simulink model "RingSpinning_Bearing_DigitalTwin_Modely"  (R2025b)
settings: Solver=ode4  StartTime=0.0  StopTime=10  FixedStep=7.8125e-05  RelTol=1e-3
undefined symbols (not defined in the file): ambient_temp, bpfo_hz, Cth, damping_ratio, fault_severity, imbalance_amp, initial_temp, Kth, misalignment_amp, omega, P_loss, rpm, sensor_noise_std, wn
settings Model: Creator=Dhiyayanth  LastModifiedBy=Dhiyayanth

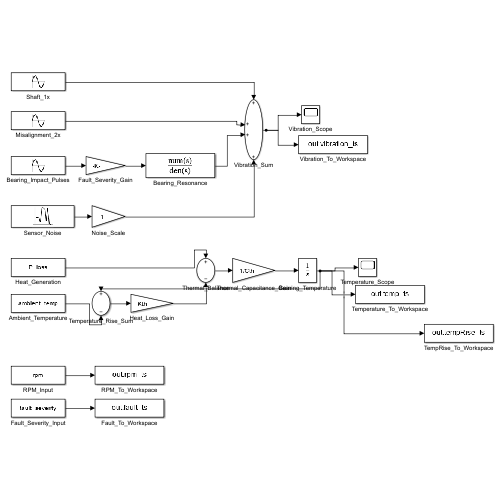
[thumbnail: Simulink's stored preview of the top-level diagram]
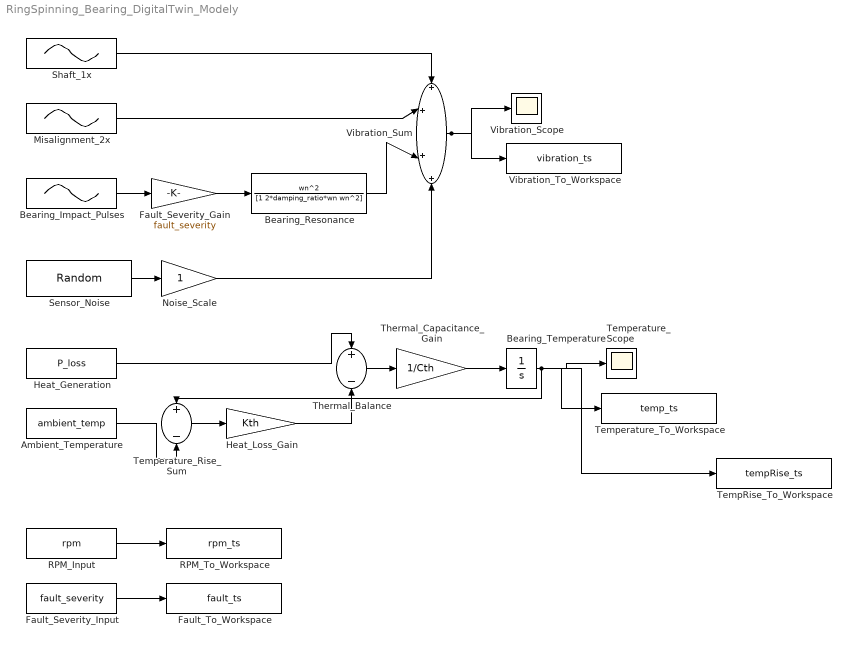
== system RingSpinning_Bearing_DigitalTwin_Modely ==
  Ambient_Temperature : Constant  Value=ambient_temp
  Bearing_Impact_Pulses : Sin  Frequency=2*pi*bpfo_hz  SampleTime=0
  Bearing_Resonance : TransferFcn  Numerator=wn^2  Denominator=[1 2*damping_ratio*wn wn^2]
  Bearing_Temperature : Integrator  InitialCondition=initial_temp
  Fault_Severity_Gain : Gain  Gain=fault_severity
  Fault_Severity_Input : Constant  Value=fault_severity
  Fault_To_Workspace : ToWorkspace  VariableName=fault_ts  SaveFormat=Timeseries  SampleTime=-1
  Heat_Generation : Constant  Value=P_loss
  Heat_Loss_Gain : Gain  Gain=Kth
  Misalignment_2x : Sin  Amplitude=misalignment_amp  Frequency=2*omega  SampleTime=0
  Noise_Scale : Gain
  RPM_Input : Constant  Value=rpm
  RPM_To_Workspace : ToWorkspace  VariableName=rpm_ts  SaveFormat=Timeseries  SampleTime=-1
  Sensor_Noise : RandomNumber  Variance=sensor_noise_std^2  Seed=1234  SampleTime=7.8125e-05
  Shaft_1x : Sin  Amplitude=imbalance_amp  Frequency=omega  SampleTime=0
  TempRise_To_Workspace : ToWorkspace  VariableName=tempRise_ts  SaveFormat=Timeseries  SampleTime=-1
  Temperature_Rise_Sum : Sum  Inputs=+-
  Temperature_Scope : Scope
  Temperature_To_Workspace : ToWorkspace  VariableName=temp_ts  SaveFormat=Timeseries  SampleTime=-1
  Thermal_Balance : Sum  Inputs=+-
  Thermal_Capacitance_Gain : Gain  Gain=1/Cth
  Vibration_Scope : Scope
  Vibration_Sum : Sum  Inputs=++++
  Vibration_To_Workspace : ToWorkspace  VariableName=vibration_ts  SaveFormat=Timeseries  SampleTime=-1
  wires:
  Shaft_1x/1 -> Vibration_Sum/1
  Misalignment_2x/1 -> Vibration_Sum/2
  Bearing_Impact_Pulses/1 -> Fault_Severity_Gain/1
  Fault_Severity_Gain/1 -> Bearing_Resonance/1
  Bearing_Resonance/1 -> Vibration_Sum/3
  Sensor_Noise/1 -> Noise_Scale/1
  Noise_Scale/1 -> Vibration_Sum/4
  Vibration_Sum/1 -> Vibration_Scope/1, Vibration_To_Workspace/1
  Bearing_Temperature/1 -> Temperature_Rise_Sum/1, Temperature_Scope/1, Temperature_To_Workspace/1, TempRise_To_Workspace/1
  Ambient_Temperature/1 -> Temperature_Rise_Sum/2
  Temperature_Rise_Sum/1 -> Heat_Loss_Gain/1
  Heat_Generation/1 -> Thermal_Balance/1
  Heat_Loss_Gain/1 -> Thermal_Balance/2
  Thermal_Balance/1 -> Thermal_Capacitance_Gain/1
  Thermal_Capacitance_Gain/1 -> Bearing_Temperature/1
  RPM_Input/1 -> RPM_To_Workspace/1
  Fault_Severity_Input/1 -> Fault_To_Workspace/1
